simulink model "foc_1"  (R2022b)
settings: Solver=VariableStepAuto  StartTime=0.0  StopTime=0.5  RelTol=1e-3
InitFcn:
  | SPEED_PI_P=0.003
  | SPEED_PI_I=5
  | SPEED_PI_UP_LIMIT = 5.0
  | SPEED_PI_LOW_LIMIT = -5.0
  | SPEED_PI_KB = 0.015
  | D_PI_P = 1.4
  | D_PI_I = 600
  | D_PI_UP_LIMIT = 24.0
  | D_PI_LOW_LIMIT = -24.0
  | D_PI_KB = 15
  | Q_PI_P = 1.4
  | Q_PI_I = 600
  | Q_PI_UP_LIMIT = 24.0
  | Q_PI_LOW_LIMIT = -24.0
  | Q_PI_KB = 15
  | Pn = 1.0
  | Ld = 1.4e-3
  | Lq = 1.4e-3
  | Flux=0.034182
  | R = 0.6
  | J = 1.1e-5
  | DK = 50
libraries: simulink x2, slpidlib x2, spsDCVoltageSourceLib x1, spsGroundLib x1, spsPermanentMagnetSynchronousMachineLib x1, spsThreePhaseVIMeasurementLib x1, spsUniversalBridgeLib x1, sps_lib x1
settings Model: Creator=15403  LastModifiedBy=15403

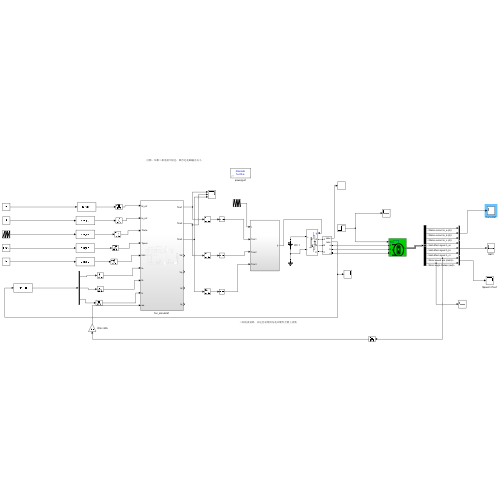
[thumbnail: Simulink's stored preview of the top-level diagram]
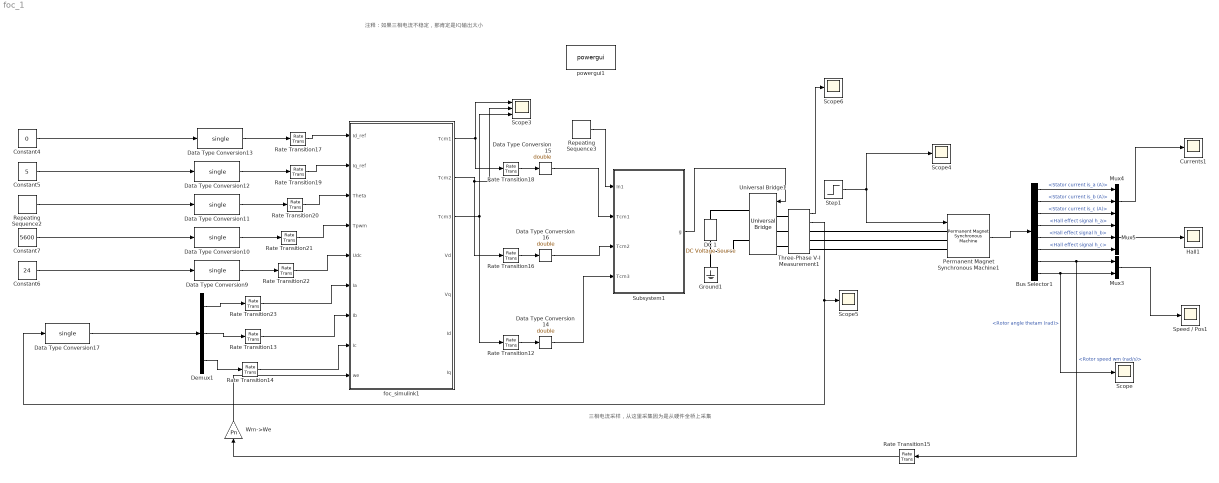
== system foc_1 ==
  note: 注释：如果三相电流不稳定，那肯定是IQ输出太小
  note: 三相电流采样，从这里采集因为是从硬件全桥上采集
  Bus Selector1 : BusSelector  OutputSignals=Stator current is_a (A),Stator current is_b (A),Stator current is_c (A),Hall effect signal h_a,Hall effect signal h_b,Hall effect signal h_c,Rotor speed wm (rad/s),Rotor angle thetam (rad)
  Constant4 : Constant  Value=0
  Constant5 : Constant  Value=5
  Constant6 : Constant  Value=24
  Constant7 : Constant  Value=5600
  Currents1 : Scope
  DC 1 : spsDCVoltageSourceLib/DC Voltage Source  Amplitude=24  Measurements=None
  Data Type Conversion{9..13,17} (6 alike) : DataTypeConversion  OutDataTypeStr=single  SaturateOnIntegerOverflow=off  RndMeth=Floor
  Data Type Conversion14 : DataTypeConversion  OutDataTypeStr=double  SaturateOnIntegerOverflow=off  RndMeth=Floor
  Data Type Conversion15 : DataTypeConversion  OutDataTypeStr=double  SaturateOnIntegerOverflow=off  RndMeth=Floor
  Data Type Conversion16 : DataTypeConversion  OutDataTypeStr=double  SaturateOnIntegerOverflow=off  RndMeth=Floor
  Demux1 : Demux  Outputs=3
  Ground1 : spsGroundLib/Ground  LConnTagsString=a
  Hall1 : Scope
  Mux3 : Mux  Inputs=2
  Mux4 : Mux  Inputs=3
  Mux5 : Mux  Inputs=3
  Permanent Magnet Synchronous Machine1 : spsPermanentMagnetSynchronousMachineLib/Permanent Magnet Synchronous Machine  NbPhases=3  FluxDistribution=Sinusoidal  RotorType=Round  MechanicalLoad=Torque Tm  PresetModel=No  ShowDetailedParameters=on  MeasurementBus=off  Resistance=0.6  Inductance=8.5e-3  dqInductances=[8.5e-3, 8.5e-3]  La=1.4e-3  MachineConstant=Flux linkage established by magnets (V.s)  Flux=0.034182  VoltageCst=6.1999  TorqueCst=0.051273  Flat=120  Mechanical=[1.1e-5,1e-4,1,0.02]  PolePairs=4  InitialConditions=[0,0, 0,0]  InitialConditions5ph=[0 0 0 0 0 0]  RefAngle=Aligned with phase A axis (original Park)  IterativeDiscreteModel=Trapezoidal non iterative  TsBlock=-1  TsPowergui=0
  Rate Transition{12..23} (12 alike) : RateTransition
  Repeating Sequence2 : simulink/Sources/Repeating Sequence  rep_seq_t=[0 0.1]  rep_seq_y=[0 2 * pi]
  Repeating Sequence3 : simulink/Sources/Repeating Sequence  rep_seq_t=[0 1/15000 2/15000]  rep_seq_y=[0 2800 0]
  Scope{,4..6} (4 alike) : Scope
  Scope3 : Scope  NumInputPorts=3
  Speed / Pos1 : Scope
  Step1 : Step  Time=0  After=0  SampleTime=0
  Subsystem1 : Subsystem
  Three-Phase V-I Measurement1 : spsThreePhaseVIMeasurementLib/Three-Phase V-I Measurement  VoltageMeasurement=phase-to-ground  SetLabelV=off  LabelV=Vabc  Vpu=off  VpuLL=off  CurrentMeasurement=yes  SetLabelI=off  LabelI=Iabc  Ipu=off  Pbase=100e6  Vbase=500e3  OutputType=Complex  PhasorSimulation=off  PSBequivalent=0
  Universal Bridge1 : spsUniversalBridgeLib/Universal Bridge  Arms=3  SnubberResistance=1e5  SnubberCapacitance=inf  Device=IGBT / Diodes  Ron=1e-3  Lon=0  ForwardVoltages="[  0  0  ]"  ForwardVoltage=0  GTOparameters=[ 10e-6 , 20e-6 ]  IGBTparameters=[ 1e-6 , 2e-6 ]  Measurements=None  Measurements_2=None  converterType=Rectifier
  Wm->We : Gain  Gain=Pn
  foc_simulink1 : Subsystem
  powergui1 : sps_lib/powergui  Priority=1  SimulationMode=Discrete  SampleTime=0.000001  frequency=60  Iterations=50  frequencyindice=0  Pbase=100e6  ErrMax=1e-4  UnitsV=kV  UnitsW=MW  buscounter=0  FunctionMessages=off  echomessages=off  EnableUseOfTLC=off  CurrentSourceSwitches=off  DisableSnubberDevices=off  DisableRonSwitches=off  DisableVfSwitches=off  DisplayEquations=off  AutomaticDiscreteSolvers=off  SolverType=Tustin/Backward Euler (TBE)  Interpol=off  ExternalGateDelay=off  methode=off  Ts=100  x0status=blocks  SPID=on  SwTol=0  HookPort=off  NonlinearTolerance=1e-4  nMaxIteration=100  ContinueOnMaxIteration=off  RestoreLinks=warning  ResistiveCurrentMeasurement=off  Frange=[0:2:500]  Ylog=off  Xlog=on  ShowGrid=off  save=off  variable=ZData  structure=0  ZoomFFT=off  StartTime=0.0  cycles=1  DisplayStyle=1  fundamental=60  FreqAxis=off  MaxFrequency=1000  frequencyindicesteady=1  RmsSteady=1  display=off
  wires:
  Permanent Magnet Synchronous Machine1/1 -> Bus Selector1/1
  Three-Phase V-I Measurement1/1 -> Scope6/1
  Demux1/3 -> Rate Transition14/1
  Rate Transition13/1 -> foc_simulink1/7(Ib)
  Bus Selector1/3 -> Mux4/3  "<Stator current is_c (A)>"
  Mux4/1 -> Currents1/1
  Mux5/1 -> Hall1/1
  Data Type Conversion10/1 -> Rate Transition21/1
  Bus Selector1/5 -> Mux5/2  "<Hall effect signal h_b>"
  Demux1/2 -> Rate Transition13/1
  Step1/1 -> Permanent Magnet Synchronous Machine1/1, Scope4/1
  Data Type Conversion9/1 -> Rate Transition22/1
  Three-Phase V-I Measurement1/2 -> Scope5/1, Data Type Conversion17/1
  foc_simulink1/3(Tcm3) -> Rate Transition12/1, Scope3/3
  foc_simulink1/1(Tcm1) -> Rate Transition18/1, Scope3/1
  Subsystem1/1(g) -> Universal Bridge1/1
  Data Type Conversion11/1 -> Rate Transition20/1
  Rate Transition19/1 -> foc_simulink1/2(Iq_ref)
  Mux3/1 -> Speed / Pos1/1
  Bus Selector1/1 -> Mux4/1  "<Stator current is_a (A)>"
  Rate Transition23/1 -> foc_simulink1/6(Ia)
  Data Type Conversion17/1 -> Demux1/1
  Bus Selector1/4 -> Mux5/1  "<Hall effect signal h_a>"
  Constant7/1 -> Data Type Conversion10/1
  Bus Selector1/2 -> Mux4/2  "<Stator current is_b (A)>"
  foc_simulink1/2(Tcm2) -> Rate Transition16/1, Scope3/2
  Rate Transition21/1 -> foc_simulink1/4(Tpwm)
  Constant6/1 -> Data Type Conversion9/1
  Wm->We/1 -> foc_simulink1/9(we)
  Rate Transition12/1 -> Data Type Conversion14/1
  Rate Transition17/1 -> foc_simulink1/1(Id_ref)
  Rate Transition15/1 -> Wm->We/1
  Constant4/1 -> Data Type Conversion13/1
  Rate Transition18/1 -> Data Type Conversion15/1
  Bus Selector1/6 -> Mux5/3  "<Hall effect signal h_c>"
  Rate Transition20/1 -> foc_simulink1/3(Theta)
  Data Type Conversion12/1 -> Rate Transition19/1
  Bus Selector1/8 -> Scope/1, Mux3/2  "<Rotor angle thetam (rad)>"
  Rate Transition14/1 -> foc_simulink1/8(Ic)
  Rate Transition16/1 -> Data Type Conversion16/1
  Data Type Conversion13/1 -> Rate Transition17/1
  Data Type Conversion16/1 -> Subsystem1/3(Tcm2)
  Data Type Conversion15/1 -> Subsystem1/2(Tcm1)
  Data Type Conversion14/1 -> Subsystem1/4(Tcm3)
  Rate Transition22/1 -> foc_simulink1/5(Udc)
  Demux1/1 -> Rate Transition23/1
  Bus Selector1/7 -> Rate Transition15/1, Mux3/1  "<Rotor speed wm (rad/s)>"
  Constant5/1 -> Data Type Conversion12/1
  Repeating Sequence3/1 -> Subsystem1/1(In1)
  Repeating Sequence2/1 -> Data Type Conversion11/1
  connections:
  DC 1/LConn1 -- Universal Bridge1/RConn2 -- Ground1/LConn1
  Universal Bridge1/LConn1 -- Three-Phase V-I Measurement1/LConn1
  Universal Bridge1/LConn2 -- Three-Phase V-I Measurement1/LConn2
  Three-Phase V-I Measurement1/RConn2 -- Permanent Magnet Synchronous Machine1/LConn2
  DC 1/RConn1 -- Universal Bridge1/RConn1
  Three-Phase V-I Measurement1/RConn3 -- Permanent Magnet Synchronous Machine1/LConn3
  Universal Bridge1/LConn3 -- Three-Phase V-I Measurement1/LConn3
  Three-Phase V-I Measurement1/RConn1 -- Permanent Magnet Synchronous Machine1/LConn1

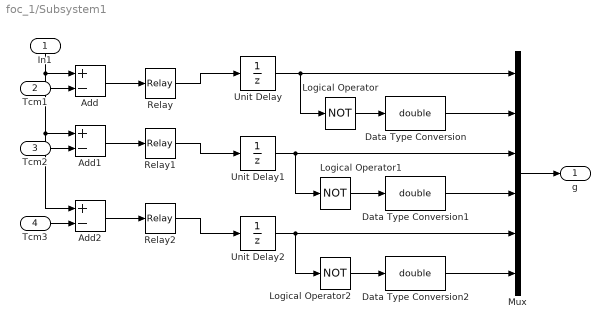
== system foc_1/Subsystem1 ==
  In1 : Inport
  Tcm1 : Inport  Port=2
  Tcm2 : Inport  Port=3
  Tcm3 : Inport  Port=4
  Add : Sum  Inputs=+-
  Add1 : Sum  Inputs=+-
  Add2 : Sum  Inputs=+-
  Data Type Conversion : DataTypeConversion  OutDataTypeStr=double  SaturateOnIntegerOverflow=off  RndMeth=Floor
  Data Type Conversion1 : DataTypeConversion  OutDataTypeStr=double  SaturateOnIntegerOverflow=off  RndMeth=Floor
  Data Type Conversion2 : DataTypeConversion  OutDataTypeStr=double  SaturateOnIntegerOverflow=off  RndMeth=Floor
  Logical Operator : Logic  Operator=NOT  AllPortsSameDT=off  OutDataTypeStr=boolean
  Logical Operator1 : Logic  Operator=NOT  AllPortsSameDT=off  OutDataTypeStr=boolean
  Logical Operator2 : Logic  Operator=NOT  AllPortsSameDT=off  OutDataTypeStr=boolean
  Mux : Mux  Inputs=6
  Relay : Relay  OffSwitchValue=-eps
  Relay1 : Relay  OffSwitchValue=-eps
  Relay2 : Relay  OffSwitchValue=-eps
  Unit Delay : UnitDelay  SampleTime=-1  HasFrameUpgradeWarning=on
  Unit Delay1 : UnitDelay  SampleTime=-1  HasFrameUpgradeWarning=on
  Unit Delay2 : UnitDelay  SampleTime=-1  HasFrameUpgradeWarning=on
  g : Outport  VectorParamsAs1DForOutWhenUnconnected=off
  wires:
  Tcm3/1 -> Add2/2
  Tcm2/1 -> Add1/2
  Tcm1/1 -> Add/2
  Relay2/1 -> Unit Delay2/1
  Relay1/1 -> Unit Delay1/1
  Relay/1 -> Unit Delay/1
  Unit Delay2/1 -> Mux/5, Logical Operator2/1
  Unit Delay1/1 -> Mux/3, Logical Operator1/1
  Unit Delay/1 -> Logical Operator/1, Mux/1
  Mux/1 -> g/1
  Data Type Conversion/1 -> Mux/2
  Data Type Conversion1/1 -> Mux/4
  Data Type Conversion2/1 -> Mux/6
  Logical Operator2/1 -> Data Type Conversion2/1
  Logical Operator1/1 -> Data Type Conversion1/1
  Logical Operator/1 -> Data Type Conversion/1
  Add1/1 -> Relay1/1
  Add2/1 -> Relay2/1
  Add/1 -> Relay/1
  In1/1 -> Add/1, Add2/1, Add1/1

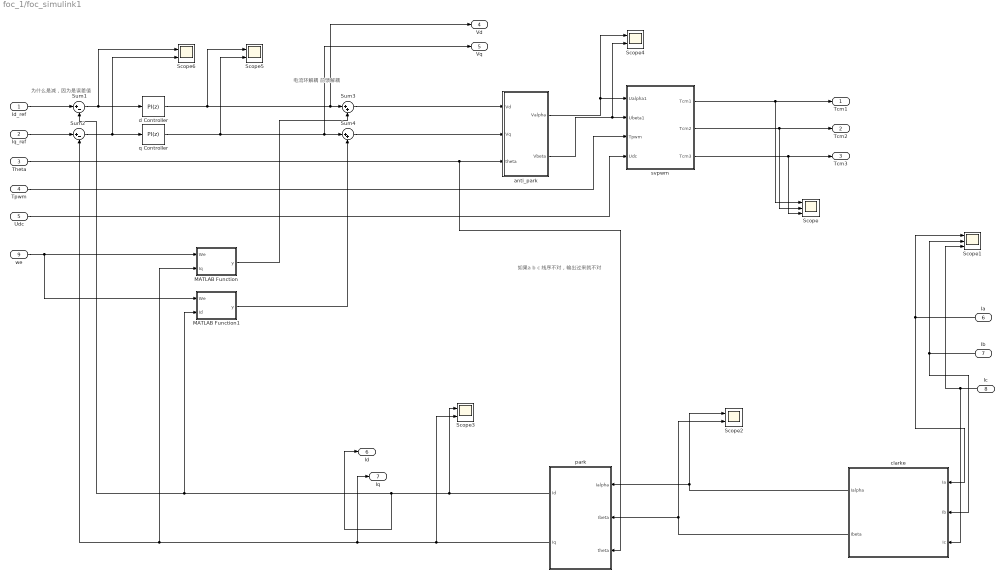
== system foc_1/foc_simulink1 ==
  note: 电流环解耦
      | 前馈解耦
  note: 为什么是减，因为是误差值
  note: 如果a b c 线序不对，输出过来就不对
  Id_ref : Inport
  Iq_ref : Inport  Port=2
  Theta : Inport  Port=3
  Tpwm : Inport  Port=4
  Udc : Inport  Port=5
  Ia : Inport  Port=6
  Ib : Inport  Port=7
  Ic : Inport  Port=8
  we : Inport  Port=9
  MATLAB Function : MATLAB Function  TreatAsAtomicUnit=on
  MATLAB Function1 : MATLAB Function  TreatAsAtomicUnit=on
  Scope : Scope  NumInputPorts=3
  Scope1 : Scope  NumInputPorts=3
  Scope{2..6} (5 alike) : Scope  NumInputPorts=2
  Sum1 : Sum  Inputs=|+-
  Sum2 : Sum  Inputs=|+-
  Sum3 : Sum  Inputs=|++
  Sum4 : Sum  Inputs=|++
  anti_park : Subsystem
  clarke : Subsystem
  d Controller : slpidlib/PID Controller  Controller=PI  Form=Parallel  TimeDomain=Discrete-time  UseExternalTs=off  SampleTime=-1  IntegratorMethod=Forward Euler  FilterMethod=Forward Euler  ControllerParametersSource=internal  P=2 * pi * R  I=2 * pi * R * R / Ld  UseKiTs=off  D=0.09  N=100  UseFilter=on  TunerSelectOption=Transfer Function Based (PID Tuner App)  InitialConditionSource=internal  InitialConditionForIntegrator=0  InitialConditionForFilter=0  DifferentiatorICPrevScaledInput=0  ExternalReset=none  TrackingMode=off  Kt=1  LimitOutput=on  SatLimitsSource=internal  UpperSaturationLimit=D_PI_UP_LIMIT  LowerSaturationLimit=D_PI_LOW_LIMIT  LinearizeAsGain=off  AntiWindupMode=back-calculation  Kb=D_PI_KB  LimitIntegrator=off  UpperIntegratorSaturationLimit=inf  LowerIntegratorSaturationLimit=-inf  PGainOutDataTypeStr=single  PProdOutDataTypeStr=single  POutMin=[]  POutMax=[]  IGainOutDataTypeStr=single  IProdOutDataTypeStr=single  IOutMin=[]  IOutMax=[]  DOutMin=[]  DOutMax=[]  NOutMin=[]  NOutMax=[]  SumOutDataTypeStr=single  SumOutMin=[]  SumOutMax=[]  SaturationOutDataTypeStr=single  SaturationOutMin=[]  SaturationOutMax=[]  PParamDataTypeStr=single  PParamMin=[]  PParamMax=[]  IParamDataTypeStr=single  IParamMin=[]  IParamMax=[]  DParamMin=[]  DParamMax=[]  NParamMin=[]  NParamMax=[]  KbParamDataTypeStr=single  KbParamMin=[]  KbParamMax=[]  KtParamMin=[]  KtParamMax=[]  KbOutDataTypeStr=single  KbOutMin=[]  KbOutMax=[]  KtOutMin=[]  KtOutMax=[]  IntegratorOutDataTypeStr=single  IntegratorOutMin=[]  IntegratorOutMax=[]  FilterOutMin=[]  FilterOutMax=[]  SumI1OutDataTypeStr=single  SumI1OutMin=[]  SumI1OutMax=[]  SumI2OutDataTypeStr=single  SumI2OutMin=[]  SumI2OutMax=[]  SumI3OutMin=[]  SumI3OutMax=[]  SumI4OutMin=[]  SumI4OutMax=[]  SumDOutMin=[]  SumDOutMax=[]  SumAccumDataTypeStr=single  SumI1AccumDataTypeStr=single  SumI2AccumDataTypeStr=single  DifferentiatorOutMin=[]  DifferentiatorOutMax=[]  FilterDiffOutCoefMin=[]  FilterDiffOutCoefMax=[]  ReciprocalOutMin=[]  ReciprocalOutMax=[]  SumDenOutMin=[]  SumDenOutMax=[]  SumNumOutMin=[]  SumNumOutMax=[]  DivideOutMin=[]  DivideOutMax=[]  UdiffTsProdOutMin=[]  UdiffTsProdOutMax=[]  NTsProdOutMin=[]  NTsProdOutMax=[]  UintegralTsProdOutMin=[]  UintegralTsProdOutMax=[]  UngainTsProdOutMin=[]  UngainTsProdOutMax=[]  ClampingZeroOutDataTypeStr=Inherit: Inherit via back propagation  ClampingZeroOutMin=[]  ClampingZeroOutMax=[]  FilterDenConstantOutDataTypeStr=Inherit: Inherit via back propagation  FilterDenConstantOutMin=[]  FilterDenConstantOutMax=[]  PCopyOutDataTypeStr=Inherit: Inherit via back propagation  PCopyOutMin=[]  PCopyOutMax=[]  NCopyOutDataTypeStr=Inherit: Inherit via back propagation  NCopyOutMin=[]  NCopyOutMax=[]  IntegratorContinuousStateAttributes=''  IntegratorStateIdentifier=di  IntegratorStateMustResolveToSignalObject=off  IntegratorRTWStateStorageClass=Auto  FilterContinuousStateAttributes=''  FilterStateMustResolveToSignalObject=off  FilterRTWStateStorageClass=Auto  ParallelPVariant=InternalParameters  IdealPVariant=Disabled  IVariant=InternalParameters  DVariant=Disabled  IntegratorVariant=Discrete  SatVariant=Enabled  AWVariant=BackCalculation  PCopyVariant=Disabled  TRVariant=Disabled  FdbkBlocksVariant=Forward  IdealPFdbkVariant=Disabled  SatFdbkVariant=Disabled  DerivativeFilterVariant=Disabled  NVariant=Disabled  NCopyVariant=Disabled_SignalSpec  FilterICVariant=Disabled  IntegratorICVariant=InternalICs  ExternalResetVariant=Disabled  TRSumVariant=Passthrough  SumFdbkVariant=Disabled  SumVariant=Sum_PI  TsampFilterVariant=InternalTs  TsampNgainVariant=Passthrough  TsampIntegralVariant=Passthrough  ExternalSaturationOutDataTypeStr=Inherit: Same as second input
  park : Subsystem
  q Controller : slpidlib/PID Controller  Controller=PI  Form=Parallel  TimeDomain=Discrete-time  UseExternalTs=off  SampleTime=-1  IntegratorMethod=Forward Euler  FilterMethod=Forward Euler  ControllerParametersSource=internal  P=2 * pi * R  I=2 * pi * R * R / Lq  UseKiTs=off  D=0.09  N=100  UseFilter=on  TunerSelectOption=Transfer Function Based (PID Tuner App)  InitialConditionSource=internal  InitialConditionForIntegrator=0  InitialConditionForFilter=0  DifferentiatorICPrevScaledInput=0  ExternalReset=none  TrackingMode=off  Kt=1  LimitOutput=on  SatLimitsSource=internal  UpperSaturationLimit=Q_PI_UP_LIMIT  LowerSaturationLimit=Q_PI_LOW_LIMIT  LinearizeAsGain=off  AntiWindupMode=back-calculation  Kb=Q_PI_KB  LimitIntegrator=off  UpperIntegratorSaturationLimit=inf  LowerIntegratorSaturationLimit=-inf  PGainOutDataTypeStr=single  PProdOutDataTypeStr=single  POutMin=[]  POutMax=[]  IGainOutDataTypeStr=single  IProdOutDataTypeStr=single  IOutMin=[]  IOutMax=[]  DOutMin=[]  DOutMax=[]  NOutMin=[]  NOutMax=[]  SumOutDataTypeStr=single  SumOutMin=[]  SumOutMax=[]  SaturationOutDataTypeStr=single  SaturationOutMin=[]  SaturationOutMax=[]  PParamDataTypeStr=single  PParamMin=[]  PParamMax=[]  IParamDataTypeStr=single  IParamMin=[]  IParamMax=[]  DParamMin=[]  DParamMax=[]  NParamMin=[]  NParamMax=[]  KbParamDataTypeStr=single  KbParamMin=[]  KbParamMax=[]  KtParamMin=[]  KtParamMax=[]  KbOutDataTypeStr=single  KbOutMin=[]  KbOutMax=[]  KtOutMin=[]  KtOutMax=[]  IntegratorOutDataTypeStr=single  IntegratorOutMin=[]  IntegratorOutMax=[]  FilterOutMin=[]  FilterOutMax=[]  SumI1OutDataTypeStr=single  SumI1OutMin=[]  SumI1OutMax=[]  SumI2OutDataTypeStr=single  SumI2OutMin=[]  SumI2OutMax=[]  SumI3OutMin=[]  SumI3OutMax=[]  SumI4OutMin=[]  SumI4OutMax=[]  SumDOutMin=[]  SumDOutMax=[]  SumAccumDataTypeStr=single  SumI1AccumDataTypeStr=single  SumI2AccumDataTypeStr=single  DifferentiatorOutMin=[]  DifferentiatorOutMax=[]  FilterDiffOutCoefMin=[]  FilterDiffOutCoefMax=[]  ReciprocalOutMin=[]  ReciprocalOutMax=[]  SumDenOutMin=[]  SumDenOutMax=[]  SumNumOutMin=[]  SumNumOutMax=[]  DivideOutMin=[]  DivideOutMax=[]  UdiffTsProdOutMin=[]  UdiffTsProdOutMax=[]  NTsProdOutMin=[]  NTsProdOutMax=[]  UintegralTsProdOutMin=[]  UintegralTsProdOutMax=[]  UngainTsProdOutMin=[]  UngainTsProdOutMax=[]  ClampingZeroOutDataTypeStr=Inherit: Inherit via back propagation  ClampingZeroOutMin=[]  ClampingZeroOutMax=[]  FilterDenConstantOutDataTypeStr=Inherit: Inherit via back propagation  FilterDenConstantOutMin=[]  FilterDenConstantOutMax=[]  PCopyOutDataTypeStr=Inherit: Inherit via back propagation  PCopyOutMin=[]  PCopyOutMax=[]  NCopyOutDataTypeStr=Inherit: Inherit via back propagation  NCopyOutMin=[]  NCopyOutMax=[]  IntegratorContinuousStateAttributes=''  IntegratorStateIdentifier=qi  IntegratorStateMustResolveToSignalObject=off  IntegratorRTWStateStorageClass=Auto  FilterContinuousStateAttributes=''  FilterStateMustResolveToSignalObject=off  FilterRTWStateStorageClass=Auto  ParallelPVariant=InternalParameters  IdealPVariant=Disabled  IVariant=InternalParameters  DVariant=Disabled  IntegratorVariant=Discrete  SatVariant=Enabled  AWVariant=BackCalculation  PCopyVariant=Disabled  TRVariant=Disabled  FdbkBlocksVariant=Forward  IdealPFdbkVariant=Disabled  SatFdbkVariant=Disabled  DerivativeFilterVariant=Disabled  NVariant=Disabled  NCopyVariant=Disabled_SignalSpec  FilterICVariant=Disabled  IntegratorICVariant=InternalICs  ExternalResetVariant=Disabled  TRSumVariant=Passthrough  SumFdbkVariant=Disabled  SumVariant=Sum_PI  TsampFilterVariant=InternalTs  TsampNgainVariant=Passthrough  TsampIntegralVariant=Passthrough  ExternalSaturationOutDataTypeStr=Inherit: Same as second input
  svpwm : Subsystem
  Tcm1 : Outport
  Tcm2 : Outport  Port=2
  Tcm3 : Outport  Port=3
  Vd : Outport  Port=4
  Vq : Outport  Port=5
  Id : Outport  Port=6
  Iq : Outport  Port=7
  wires:
  Theta/1 -> anti_park/3(theta), park/3(theta)
  Udc/1 -> svpwm/4(Udc)
  Tpwm/1 -> svpwm/3(Tpwm)
  svpwm/3(Tcm3) -> Scope/3, Tcm3/1
  anti_park/2(Vbeta) -> Scope4/2, svpwm/2(Ubeta1)
  svpwm/1(Tcm1) -> Scope/1, Tcm1/1
  svpwm/2(Tcm2) -> Scope/2, Tcm2/1
  anti_park/1(Valpha) -> Scope4/1, svpwm/1(Ualpha1)
  clarke/2(Ibeta) -> Scope2/2, park/2(Ibeta)
  clarke/1(Ialpha) -> Scope2/1, park/1(Ialpha)
  Ia/1 -> clarke/1(Ia), Scope1/1
  Ib/1 -> clarke/2(Ib), Scope1/2
  Ic/1 -> Scope1/3, clarke/3(Ic)
  park/1(Id) -> Scope3/1, Id/1, MATLAB Function1/2(Id), Sum1/2
  park/2(Iq) -> Scope3/2, Iq/1, MATLAB Function/2(Iq), Sum2/2
  Iq_ref/1 -> Sum2/1
  Sum2/1 -> Scope6/2, q Controller/1
  q Controller/1 -> Vq/1, Sum4/1, Scope5/2
  Id_ref/1 -> Sum1/1
  Sum1/1 -> Scope6/1, d Controller/1
  d Controller/1 -> Vd/1, Sum3/1, Scope5/1
  Sum3/1 -> anti_park/1(Vd)
  Sum4/1 -> anti_park/2(Vq)
  we/1 -> MATLAB Function1/1(We), MATLAB Function/1(We)
  MATLAB Function/1(y) -> Sum3/2
  MATLAB Function1/1(y) -> Sum4/2

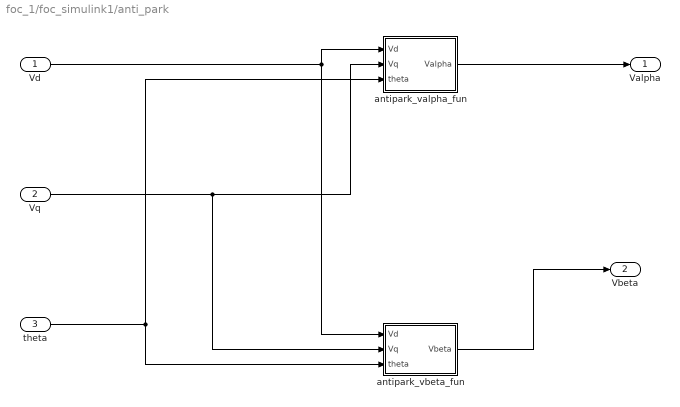
== system foc_1/foc_simulink1/anti_park ==
  Vd : Inport
  Vq : Inport  Port=2
  theta : Inport  Port=3
  antipark_valpha_fun : MATLAB Function  TreatAsAtomicUnit=on
  antipark_vbeta_fun : MATLAB Function  TreatAsAtomicUnit=on
  Valpha : Outport
  Vbeta : Outport  Port=2
  wires:
  antipark_valpha_fun/1(Valpha) -> Valpha/1
  antipark_vbeta_fun/1(Vbeta) -> Vbeta/1
  Vd/1 -> antipark_valpha_fun/1(Vd), antipark_vbeta_fun/1(Vd)
  Vq/1 -> antipark_valpha_fun/2(Vq), antipark_vbeta_fun/2(Vq)
  theta/1 -> antipark_valpha_fun/3(theta), antipark_vbeta_fun/3(theta)

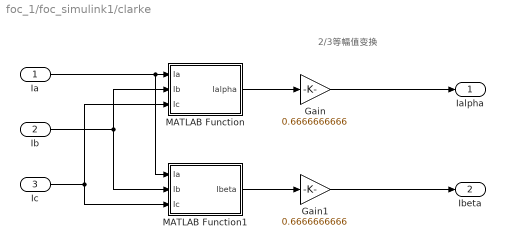
== system foc_1/foc_simulink1/clarke ==
  note: 2/3等幅值变换
  Ia : Inport
  Ib : Inport  Port=2
  Ic : Inport  Port=3
  Gain : Gain  Gain=0.6666666666  OutDataTypeStr=single
  Gain1 : Gain  Gain=0.6666666666  OutDataTypeStr=single
  MATLAB Function : MATLAB Function  TreatAsAtomicUnit=on
  MATLAB Function1 : MATLAB Function  TreatAsAtomicUnit=on
  Ialpha : Outport
  Ibeta : Outport  Port=2
  wires:
  Ia/1 -> MATLAB Function1/1(Ia), MATLAB Function/1(Ia)
  MATLAB Function/1(Ialpha) -> Gain/1
  Gain1/1 -> Ibeta/1
  Ib/1 -> MATLAB Function1/2(Ib), MATLAB Function/2(Ib)
  Ic/1 -> MATLAB Function/3(Ic), MATLAB Function1/3(Ic)
  MATLAB Function1/1(Ibeta) -> Gain1/1
  Gain/1 -> Ialpha/1

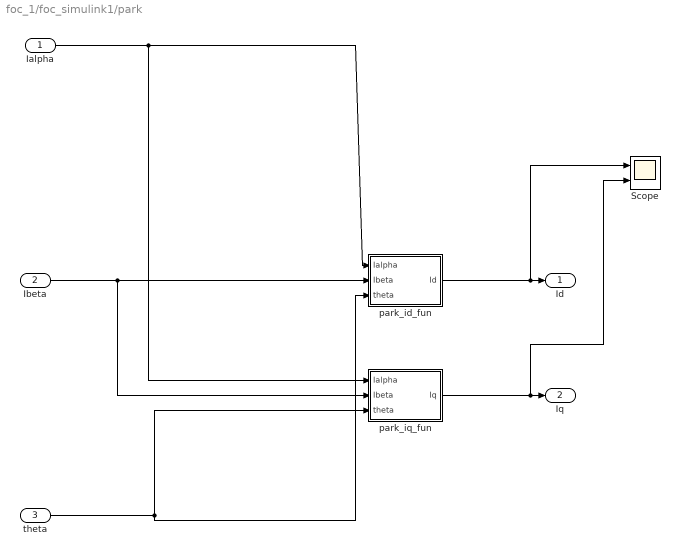
== system foc_1/foc_simulink1/park ==
  Ialpha : Inport
  Ibeta : Inport  Port=2
  theta : Inport  Port=3
  Scope : Scope  NumInputPorts=2
  park_id_fun : MATLAB Function  TreatAsAtomicUnit=on
  park_iq_fun : MATLAB Function  TreatAsAtomicUnit=on
  Id : Outport
  Iq : Outport  Port=2
  wires:
  theta/1 -> park_id_fun/3(theta), park_iq_fun/3(theta)
  Ibeta/1 -> park_id_fun/2(Ibeta), park_iq_fun/2(Ibeta)
  park_iq_fun/1(Iq) -> Scope/2, Iq/1
  park_id_fun/1(Id) -> Scope/1, Id/1
  Ialpha/1 -> park_id_fun/1(Ialpha), park_iq_fun/1(Ialpha)

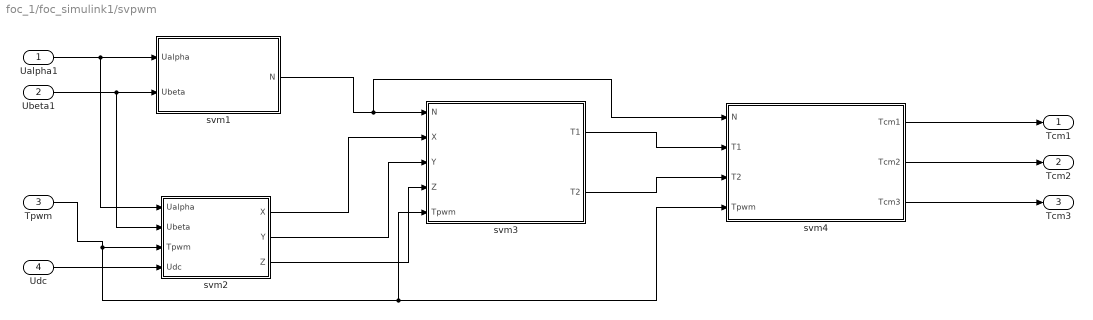
== system foc_1/foc_simulink1/svpwm ==
  Ualpha1 : Inport
  Ubeta1 : Inport  Port=2
  Tpwm : Inport  Port=3
  Udc : Inport  Port=4
  svm1 : MATLAB Function  TreatAsAtomicUnit=on
  svm2 : MATLAB Function  TreatAsAtomicUnit=on
  svm3 : MATLAB Function  TreatAsAtomicUnit=on
  svm4 : MATLAB Function  TreatAsAtomicUnit=on
  Tcm1 : Outport
  Tcm2 : Outport  Port=2
  Tcm3 : Outport  Port=3
  wires:
  svm4/2(Tcm2) -> Tcm2/1
  Tpwm/1 -> svm4/4(Tpwm), svm3/5(Tpwm), svm2/3(Tpwm)
  svm1/1(N) -> svm4/1(N), svm3/1(N)
  Udc/1 -> svm2/4(Udc)
  svm4/3(Tcm3) -> Tcm3/1
  svm3/1(T1) -> svm4/2(T1)
  Ualpha1/1 -> svm2/1(Ualpha), svm1/1(Ualpha)
  svm3/2(T2) -> svm4/3(T2)
  Ubeta1/1 -> svm2/2(Ubeta), svm1/2(Ubeta)
  svm4/1(Tcm1) -> Tcm1/1
  svm2/1(X) -> svm3/2(X)
  svm2/3(Z) -> svm3/4(Z)
  svm2/2(Y) -> svm3/3(Y)

== matlab function foc_1/foc_simulink1/svpwm/svm3 ==
  data: N input; T1 output; X input; Y input; Z input; Tpwm input; T2 output
function [T1, T2] = fcn(N, X, Y, Z, Tpwm)

T1 = single(0);
T2 = single(0);

if N == 1
    T1 = Z;
    T2 = Y;
elseif N == 2
    T1 = Y;
    T2 = -X;
elseif N == 3
    T1 = -Z;
    T2 = X;
elseif N == 4
    T1 = -X;
    T2 = Z;
elseif N == 5
    T1 = X;
    T2 = -Y;
elseif N == 6
    T1 = -Y;
    T2 = -Z;
end

== matlab function foc_1/foc_simulink1/svpwm/svm4 ==
  data: N input; Tcm1 output; T1 input; T2 input; Tpwm input; Tcm2 output; Tcm3 output
function [Tcm1, Tcm2, Tcm3] = fcn(N, T1, T2, Tpwm)

Tcm1 = single(0);
Tcm2 = single(0);
Tcm3 = single(0);


if N == 1
    Tcm1 = (Tpwm + T1 - T2) / 4;
    Tcm2 = (Tpwm - T1 - T2) / 4;
    Tcm3 = (Tpwm + T1 + T2) / 4;
elseif N == 2
    Tcm1 = (Tpwm - T1 - T2) / 4;
    Tcm2 = (Tpwm + T1 + T2) / 4;
    Tcm3 = (Tpwm + T1 - T2) / 4;
elseif N == 3
    Tcm1 = (Tpwm - T1 - T2) / 4;
    Tcm2 = (Tpwm + T1 - T2) / 4;
    Tcm3 = (Tpwm + T1 + T2) / 4;
elseif N == 4
    Tcm1 = (Tpwm + T1 + T2) / 4;
    Tcm2 = (Tpwm + T1 - T2) / 4;
    Tcm3 = (Tpwm - T1 - T2) / 4;
elseif N == 5
    Tcm1 = (Tpwm + T1 + T2) / 4;
    Tcm2 = (Tpwm - T1 - T2) / 4;
    Tcm3 = (Tpwm + T1 - T2) / 4;
elseif N == 6
    Tcm1 = (Tpwm + T1 - T2) / 4;
    Tcm2 = (Tpwm + T1 + T2) / 4;
    Tcm3 = (Tpwm - T1 - T2) / 4;
end

== matlab function foc_1/foc_simulink1/MATLAB Function ==
  data: We input; y output; Iq input
function y = fcn(We, Iq)

% y = -We * Lq * Iq;
y = -We * 1.4e-3 * Iq;

== matlab function foc_1/foc_simulink1/MATLAB Function1 ==
  data: We input; y output; Id input
function y = fcn(We, Id)

% y = We * (Flux + Ld * Id);  
y = We * (0.034182 + 1.4e-3 * Id);

== matlab function foc_1/foc_simulink1/anti_park/antipark_valpha_fun ==
  data: Vd input; Valpha output; Vq input; theta input
function Valpha = fcn(Vd, Vq, theta)

Valpha = Vd * cos(theta) - Vq * sin(theta);

== matlab function foc_1/foc_simulink1/anti_park/antipark_vbeta_fun ==
  data: Vd input; Vbeta output; Vq input; theta input
function Vbeta = fcn(Vd, Vq, theta)

Vbeta = Vd * sin(theta) + Vq * cos(theta);

== matlab function foc_1/foc_simulink1/clarke/MATLAB Function ==
  data: Ia input; Ialpha output; Ib input; Ic input
function Ialpha = fcn(Ia, Ib, Ic)

Ialpha = 3/2 * Ia;

== matlab function foc_1/foc_simulink1/park/park_id_fun ==
  data: Ialpha input; Id output; Ibeta input; theta input
function Id = fcn(Ialpha, Ibeta, theta)

Id = Ialpha * cos(theta) + Ibeta * sin(theta);

== matlab function foc_1/foc_simulink1/park/park_iq_fun ==
  data: Ialpha input; Iq output; Ibeta input; theta input
function Iq = fcn(Ialpha, Ibeta, theta)
Iq = -Ialpha * sin(theta) + Ibeta * cos(theta);

== matlab function foc_1/foc_simulink1/svpwm/svm1 ==
  data: Ualpha input; N output; Ubeta input
function N = fcn(Ualpha, Ubeta)

U1 = Ubeta;
U2 = sqrt(3) * Ualpha - Ubeta;
U3 = -sqrt(3) * Ualpha - Ubeta;
A = 0;
B = 0;
C = 0;

if U1 > 0
    A = 1;
else
    A = 0;
end

if U2 > 0
    B = 1;
else
    B = 0;
end

if U3 > 0
    C = 1;
else
    C = 0;
end

N = A + 2 * B + 4 * C;

== matlab function foc_1/foc_simulink1/clarke/MATLAB Function1 ==
  data: Ia input; Ibeta output; Ib input; Ic input
function Ibeta = fcn( Ia, Ib, Ic)

Ibeta = sqrt(3)/2 * (Ia + 2 * Ib);

== matlab function foc_1/foc_simulink1/svpwm/svm2 ==
  data: Ualpha input; Ubeta input; Tpwm input; Udc input; X output; Y output; Z output
function [X, Y, Z] = fcn(Ualpha, Ubeta, Tpwm, Udc)

X = sqrt(3) * Tpwm * Ubeta / Udc;
Y = sqrt(3) * Tpwm / Udc * (sqrt(3) / 2 * Ualpha + 1 / 2 * Ubeta);
Z = sqrt(3) * Tpwm / Udc * (-sqrt(3) / 2 * Ualpha + 1 / 2 * Ubeta);
